simulink model "top_integrated_nanogrid"  (R2026a)
settings: Solver=ode23t  StopTime=1
values from neighbouring files (symbols this model uses):
  irradiance_day = pchip(t_coarse, irradiance_coarse, t_sim)    [flc_init.m]
  t_sim = linspace(0, 1.0, 1001)    [flc_init.m]
undefined symbols (not defined in the file or in its folder): DiscIntNeverNeededParam
libraries: fl_lib x19, nesl_utility x14, ee_lib x13, slpidlib x2, batteryecm_lib x1, fuzblock x1, eePwmGenerator x1
(part 1 of 2)
settings Model: Creator=user  LastModifiedBy=user

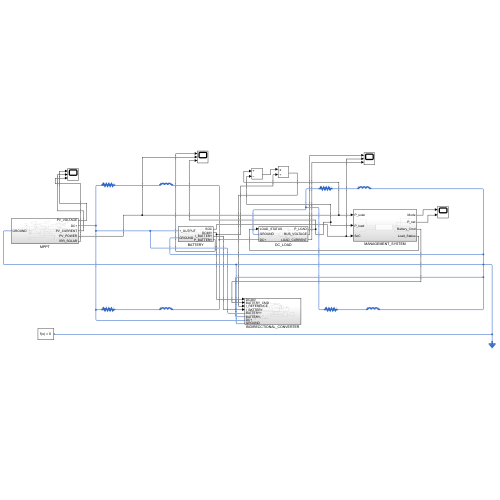
[thumbnail: Simulink's stored preview of the top-level diagram]
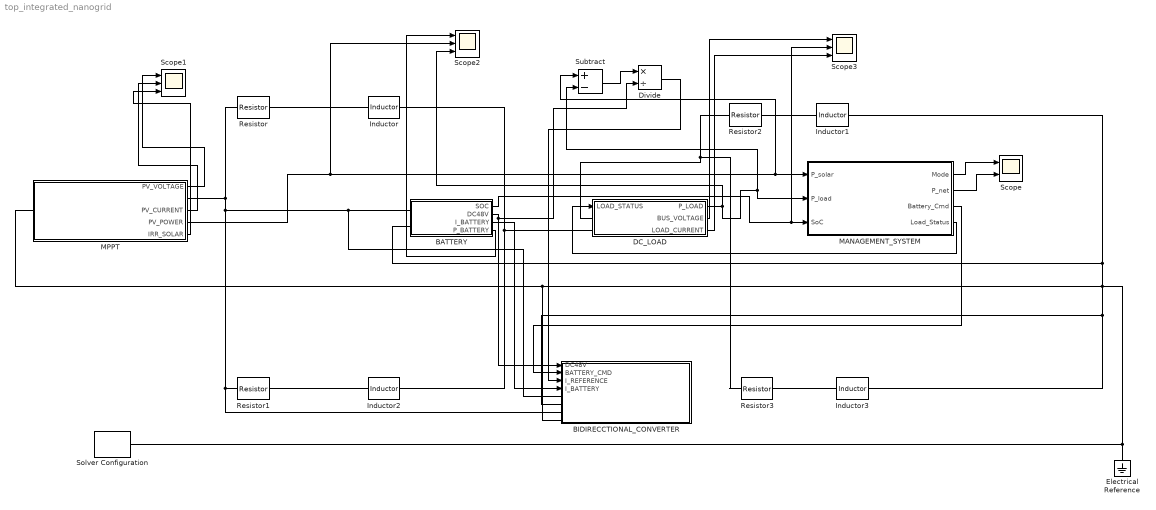
== system top_integrated_nanogrid ==
  BATTERY : Subsystem
  BIDIRECCTIONAL_CONVERTER : Subsystem
  DC_LOAD : Subsystem
  Divide : Product  Inputs=*/
  Electrical Reference : fl_lib/Electrical/Electrical Elements/Electrical Reference
  Inductor{,1..3} (4 alike) : ee_lib/Passive/Inductor  l=10e-6 H  enable_L_tol=ee.enum.toleranceApplication.none  L_tol=20  tol_distribution=ee.enum.toleranceDistribution.uniform  nSigma=4  r=0 Ohm  g=1e-9 1/Ohm  enable_operating_limits=ee.enum.enable.no  operating_limit_action=ee.enum.passive.reportOpLim.warn  max_working_current=1 A  power_rating=1 W  i_L_specify=off  i_L_priority=High  i_L=0 A  i_L_nominal_specify=off  i_L_nominal_value=1  i_L_nominal_unit=A
  MANAGEMENT_SYSTEM : Subsystem
  MPPT : Subsystem
      settings: PortSchema="{\"entries\":[{\"content\":{\"sides\":[{\"content\":{\"connectorIds\":[\"LConn1\"]},\"type\":\"ConnectorPlacement.EquallySpacedRectSide\",\"uuid\":\"0487cf4e-a869-4d13-b7ef-c52d99cbedea\"},{\"content\":{\"connectorIds\":[\"Out1\",\"RConn1\",\"Out2\",\"Out3\",\"Out4\"],\"side\":\"RIGHT\"},\"type\":\"ConnectorPlacement.EquallySpacedRectSide\",\"uuid\":\"982cd2d3-8bc2-48e7-a882-5f024f9a170e\"},{\"content\":{\"side\":\"TOP\"},\"type\":\"ConnectorPlacement.EquallySpacedRectSide\",\"uuid\":\"7eceb141-11e6-4de9-8291-895b3002810c\"}]},\"type\":\"ConnectorPlacement.EquallySpacedConnector\",\"uuid\":\"f9b56202-991f-4d6f-a8f4-53ab8bdf788c\"}],\"packageUris\":[\"http://schema.mathworks.com/mf0/Connector/R2020b\"],\"version\":\"1.0\"}"
  Resistor{,1..3} (4 alike) : fl_lib/Electrical/Electrical Elements/Resistor  R=0.23 Ohm  i_specify=off  i_priority=None  i=0 A  i_nominal_specify=off  i_nominal_value=1  i_nominal_unit=A  v_specify=off  v_priority=None  v=0 V  v_nominal_specify=off  v_nominal_value=1  v_nominal_unit=V
  Scope : Scope  NumInputPorts=2
      settings: ActiveDisplayYMinimum=-1  ActiveDisplayYMaximum=1
  Scope1 : Scope  NumInputPorts=3
      settings: ActiveDisplayYMinimum=-0.0015866090300095147  ActiveDisplayYMaximum=0.014279481270085636
  Scope2 : Scope  NumInputPorts=3
      settings: ActiveDisplayYMinimum=-1  ActiveDisplayYMaximum=1  DataLoggingVariableName=ScopeData2
  Scope3 : Scope  NumInputPorts=3
      settings: ActiveDisplayYMinimum=14.753584599444343  ActiveDisplayYMaximum=59.304634607665662  DataLoggingVariableName=ScopeData3
  Solver Configuration : nesl_utility/Solver Configuration  PhysicalDomain=network_engine_domain  SubClassName=solver  LeftPortType=input  RightPortType=generic  Tones=[]  Harmonics=[]  SimulateNoise=off  Profile=off  UseLocalSampling=off  EnableSwitchedLinearOptims=on  FrequencyDomain=off  UseCCode=off  RelTol=0.001  AbsTol=0.001  MinStep=1e-09  ToWorkspace=off  RevertToSquareIcSolve=off  NumHomotopyIterations=100  PhasorMode=off  PhasorModeNumHarmonics=1  ConsistencySolver=NEWTON_XTOL_AFTER_FTOL  CanonicalOrdering=CANONICAL  OptimizeIntermediates=OPTIMIZED  IndexReductionMethod=DerivativeReplacement  DoDC=off  ResidualTolerance=1e-09  ConsistencyTolSource=GLOBAL  ConsistencyAbsTol=0.001  ConsistencyRelTol=0.001  ConsistencyTolFactor=0.001  UseLocalSolver=off  LocalSolverChoice=NE_BACKWARD_EULER_ADVANCER  ResolveIndetEquations=on  FunctionEvalNumThread=1  LocalSolverSampleTime=0.001  DoFixedCost=off  MaxNonlinIter=3  MaxModeIter=2  ComputeImpulses=off  ImpulseIterations=2  LinearAlgebra=auto  LinearAlgebraNumThread=0  EquationFormulation=NE_TIME_EF  DelaysMemoryBudget=1024  AutomaticFiltering=on  FilteringTimeConstant=0.001  PartitionStorageMethod=AS_NEEDED  PartitionMemoryBudget=1024  PartitionMethod=ROBUST  MultibodyUseLocalSolver=off  MultibodyLocalSolverChoice=ODE1  MultibodyLocalSolverSampleTime=0.001
  Subtract : Sum  Inputs=+-
  wires:
  BATTERY/1(SOC) -> Scope3/2, MANAGEMENT_SYSTEM/3(SoC)
  MANAGEMENT_SYSTEM/4(Load_Status) -> DC_LOAD/1(LOAD_STATUS)
  MANAGEMENT_SYSTEM/1(Mode) -> Scope/1
  MANAGEMENT_SYSTEM/2(P_net) -> Scope/2
  MANAGEMENT_SYSTEM/3(Battery_Cmd) -> BIDIRECCTIONAL_CONVERTER/2(BATTERY_CMD)
  MPPT/3(PV_POWER) -> Scope2/2, Subtract/1, MANAGEMENT_SYSTEM/1(P_solar)
  DC_LOAD/1(P_LOAD) -> Subtract/2, MANAGEMENT_SYSTEM/2(P_load), Scope2/3
  Subtract/1 -> Divide/1
  BATTERY/2(DC48V) -> Divide/2, BIDIRECCTIONAL_CONVERTER/1(DC48V)
  Divide/1 -> BIDIRECCTIONAL_CONVERTER/3(I_REFERENCE)
  BATTERY/3(I_BATTERY) -> BIDIRECCTIONAL_CONVERTER/4(I_BATTERY)
  MPPT/1(PV_VOLTAGE) -> Scope1/1
  MPPT/2(PV_CURRENT) -> Scope1/2
  MPPT/4(IRR_SOLAR) -> Scope1/3
  BATTERY/4(P_BATTERY) -> Scope2/1
  DC_LOAD/2(BUS_VOLTAGE) -> Scope3/1
  DC_LOAD/3(LOAD_CURRENT) -> Scope3/3
  connections:
  Resistor/RConn1 -- Inductor/LConn1
  Resistor2/RConn1 -- Inductor1/LConn1
  Resistor1/RConn1 -- Inductor2/LConn1
  Resistor3/RConn1 -- Inductor3/LConn1
  BATTERY/LConn1 -- BIDIRECCTIONAL_CONVERTER/LConn1 -- MPPT/RConn1 -- Resistor/LConn1 -- BIDIRECCTIONAL_CONVERTER/LConn3 -- Resistor1/LConn1
  Inductor1/RConn1 -- BIDIRECCTIONAL_CONVERTER/LConn2 -- Inductor3/RConn1 -- BIDIRECCTIONAL_CONVERTER/LConn4 -- MPPT/LConn1 -- Solver Configuration/RConn1 -- Electrical Reference/LConn1 -- BATTERY/LConn2
  Inductor/RConn1 -- Inductor2/RConn1 -- DC_LOAD/LConn2
  Resistor2/LConn1 -- Resistor3/LConn1 -- DC_LOAD/LConn1

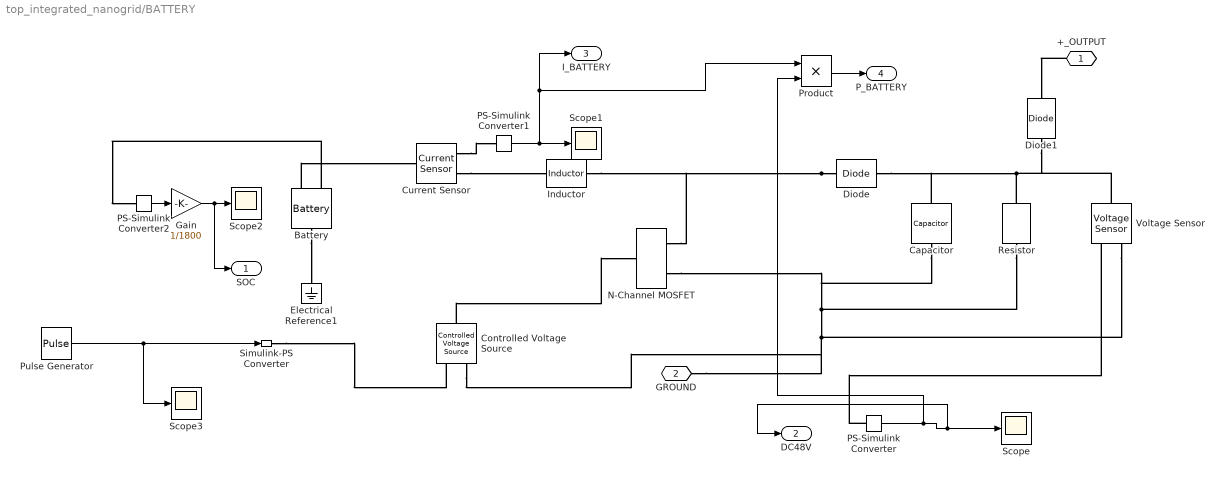
== system top_integrated_nanogrid/BATTERY ==
  Battery : batteryecm_lib/Battery  Vnom=24 V  prm_dir=simscape.enum.battery.prm_dir.enabled  R1_dis=0.001 Ohm  R1_ch=0.001 Ohm  R1=0.001 Ohm  prm_AH=simscape.enum.battery.prm_AH.finite  AH=50 A*hr  V1=11.5 V  AH1=25 A*hr  prm_R2=simscape.enum.battery.prm_R2.disabled  R2=2000 Ohm  Tmeas=298.15 K  charge_measurement_port=simscape.enum.battery.enable.yes  prm_dyn=simscape.enum.battery.prm_dyn.off  Rp1=0.005 Ohm  tau1=30 s  Rp2=0.005 Ohm  tau2=30 s  Rp3=0.005 Ohm  tau3=30 s  Rp4=0.005 Ohm  tau4=30 s  Rp5=0.005 Ohm  tau5=30 s  prm_fade=simscape.enum.battery.prm_fade.disabled  N_fade=100  AH_fade=45 A*hr  R1_fade=2.02 Ohm  R1_ch_fade=2.02 Ohm  V1_fade=10.35 V  prm_age=simscape.enum.battery.prm_age.disabled  prm_age_OCV=simscape.enum.battery.prm_age_OCV.OCV  OCV_age=0.9  SOC_age=60  Tmeas_age=298.15 K  delta_time_age_vec=[0] d  temperature_age_vec=[273] K  OCV_scaling_age=2.2134e6  OCV_offset_age=1.632e6  temp_exp_age=0.515833569 V  t_exp_age=0.75  Vnom_T2=12 V  R1_T2=2.2 Ohm  R1_T2_dis=2.2 Ohm  R1_T2_ch=2.2 Ohm  V1_T2=11.4 V  R2_T2=2200 Ohm  Rp1_T2=0.005 Ohm  tau1_T2=30 s  Rp2_T2=0.005 Ohm  tau2_T2=30 s  Rp3_T2=0.005 Ohm  tau3_T2=30 s  Rp4_T2=0.005 Ohm  tau4_T2=30 s  Rp5_T2=0.005 Ohm  tau5_T2=30 s  Tmeas2=273.15 K  thermal_port=simscape.enum.thermaleffects.omit  thermal_mass=30000 J/K  i_specify=off  i_priority=None  i=0 A  i_nominal_specify=off  i_nominal_value=1  i_nominal_unit=A  v_specify=off  v_priority=None  v=0 V  v_nominal_specify=off  v_nominal_value=1  v_nominal_unit=V  charge_specify=off  charge_priority=High  charge=50 A*hr  charge_nominal_specify=off  charge_nominal_value=1  charge_nominal_unit=A*hr  num_cycles_specify=off  num_cycles_priority=High  num_cycles=0  num_cycles_nominal_specify=off  num_cycles_nominal_value=1  num_cycles_nominal_unit=1  temperature_specify=off  temperature_priority=High  temperature=298.15 K  temperature_nominal_specify=off  temperature_nominal_value=1  temperature_nominal_unit=K
  Capacitor : fl_lib/Electrical/Electrical Elements/Capacitor  c=220 uF  r=1e-6 Ohm  g=0 1/Ohm  i_specify=off  i_priority=None  i=0 A  i_nominal_specify=off  i_nominal_value=1  i_nominal_unit=A  v_specify=off  v_priority=None  v=0 V  v_nominal_specify=off  v_nominal_value=1  v_nominal_unit=V  vc_specify=off  vc_priority=High  vc=0 V  vc_nominal_specify=off  vc_nominal_value=1  vc_nominal_unit=V
  Controlled Voltage Source : fl_lib/Electrical/Electrical Sources/Controlled Voltage Source
  Current Sensor : fl_lib/Electrical/Electrical Sensors/Current Sensor
  Diode : fl_lib/Electrical/Electrical Elements/Diode  Vf=0.7 V  Ron=0.001 Ohm  Goff=1e-8 1/Ohm  i_specify=off  i_priority=None  i=0 A  i_nominal_specify=off  i_nominal_value=1  i_nominal_unit=A  v_specify=off  v_priority=None  v=0 V  v_nominal_specify=off  v_nominal_value=1  v_nominal_unit=V
  Diode1 : ee_lib/Semiconductors & Converters/Diode  ModelType=ee.enum.diode.modelType.pwl  TableType=ee.enum.diode.tableType.IfMat  IfMat=[.07, .12, .19, 1.75, 4.24, 7.32, 11.2; .16, .3, .72, 2.14, 5.02, 8.35, 13.12] A  VfMat=[.9, 1.15, 1.25, 1.5, 1.75, 2.17, 2.6, 2.85; .58, .68, .75, 1.1, 1.38, 1.77, 2.27, 2.7] V  TjVec=[25, 125] degC  VfVec=[.5, .7, .9, 1.3, 1.7, 2.1, 2.5] V  IfVec=[.1, .2, .5, 1, 2, 4, 7, 10] A  IrMat=[1e-06, 2e-06, 5e-06, 1e-05, 2.5e-05, 5e-05, .0001; 2e-06, 5e-06, 1e-05, 4e-05, 8e-05, .0002, .0005] A  VrMat=[10, 100, 200, 250, 300, 325, 350; 10, 70, 160, 220, 270, 300, 320] V  VrVec=[10, 20, 40, 50, 70, 80, 100] V  IrVec=[1e-06, 2e-06, 5e-06, 1e-05, 2e-05, 5e-05, .0001] A  Vf=0.6 V  Ron=0.3 Ohm  Goff=1e-8 S  prmExp=ee.enum.diode.expParam.useTwo  I12=[.0137, .545] A  V12=[.6, .7] V  RS=0 Ohm  Tmeas=298.15 K  IS=1e-12 A  ec=1  I1=0.0137 A  V1=0.6 V  N_series=1  N_parallel=1  ZenerEnable=false  Rz=0.3 Ohm  BV=30 V  C_param=ee.enum.diode.capParam.fixed  CJ=0 pF  CJ0=5 pF  Vvec=[.1, 10, 100] V  Cvec=[3.5, 1, .4] pF  VJ=1 V  Mgrad=0.5  FC=0.5  Q_param=ee.enum.diode.recoveryParam.off  iRM=-7.15 A  iF=4 A  didt=-750 A/us  trr_factor=3  trr=115 ns  Qrr=150 nA*s  Vr=-600 V  Ls=150 nH  Erec=0.03 J  TT=50 ns  tau=100 ns  T_param=ee.enum.diode.temperatureParam.off  Tdevice=298.15 K  I1_T2=0.245 A  V1_T2=0.5 V  IS_T2=1.25e-7 A  Tmeas2=125 degC  XTI_param=ee.enum.diode.xtiParam.pn  XTI=3  EG_param=ee.enum.diode.egapParam.material_si  EG=1.11 eV  dBVdT=0 V/K  enable_fault_input=simscape.enum.onoff.off  i_specify=off  i_priority=None  i=0 A  i_nominal_specify=off  i_nominal_value=1  i_nominal_unit=A  v_specify=off  v_priority=None  v=0 V  v_nominal_specify=off  v_nominal_value=1  v_nominal_unit=V  v_capacitor_specify=off  v_capacitor_priority=None  v_capacitor=0 V  v_capacitor_nominal_specify=off  v_capacitor_nominal_value=1  v_capacitor_nominal_unit=V  Qj_specify=off  Qj_priority=High  Qj=0 C  Qj_nominal_specify=off  Qj_nominal_value=1  Qj_nominal_unit=C  i_diode_specify=off  i_diode_priority=None  i_diode=0 A  i_diode_nominal_specify=off  i_diode_nominal_value=1  i_diode_nominal_unit=A  v_diode_specify=off  v_diode_priority=None  v_diode=0 V  v_diode_nominal_specify=off  v_diode_nominal_value=1  v_diode_nominal_unit=V  i_capacitor_specify=off  i_capacitor_priority=None  i_capacitor=0 A  i_capacitor_nominal_specify=off  i_capacitor_nominal_value=1  i_capacitor_nominal_unit=A  fidelity_level=ee.enum.diode.fidelity.includeChargeDyn  rec_loss_model=ee.enum.diode.reverseRecoveryModelTabulateUpTo3D.fixed  ErecVal=0 J  scaleWithIandV=true  ErecMat=zeros(2, 3) J  ErecMat3D=zeros(2, 3, 2) J  TjrecVec=[298.15, 398.15] K  IfrecVec=[.1, 1, 10] A  IrecVal=10 A  VrecVal=10 V  VrecVec=[0, 100] V  tFilter=1 / 1000 / 100 s  thermal_network_parameterization=ee.enum.thermalNetworkTopology.junctionCase  Rth=[0, 10] K/W  Rth_Cauer=[1, 3, 10] K/W  Rth_Foster=[.08, .14, .22, .16] K/W  thermal_mass_parameterization=ee.enum.thermalNetwork.timeconstant  thermal_mass=[0, 1] J/K  thermal_mass_Cauer=[.1, .3, 1] J/K  thermal_mass_Foster=[.001, .005, .05, .5] J/K  thermal_time_constant=[0, 10] s  thermal_time_constant_Cauer=[1, 3, 10] s  thermal_time_constant_Foster=[7e-05, .0007, .01, .08] s  thermal_mass_initial_temperatures=[25, 25] degC  thermal_mass_initial_temperatures_Cauer=[25, 25, 25] degC  junction_thermal_mass=0.01 J/K  Tvec_initial_Foster=[25, 25, 25, 25] degC  no_thermal_network=0  junction_temperature_specify=off  junction_temperature_priority=None  junction_temperature=25 degC  junction_temperature_nominal_specify=off  junction_temperature_nominal_value=1  junction_temperature_nominal_unit=degC
  Electrical Reference1 : fl_lib/Electrical/Electrical Elements/Electrical Reference
  Gain : Gain  Gain=1/1800
  Inductor : ee_lib/Passive/Inductor  l=100 uH  enable_L_tol=ee.enum.toleranceApplication.none  L_tol=20  tol_distribution=ee.enum.toleranceDistribution.uniform  nSigma=4  r=0 Ohm  g=1e-9 1/Ohm  enable_operating_limits=ee.enum.enable.no  operating_limit_action=ee.enum.passive.reportOpLim.warn  max_working_current=1 A  power_rating=1 W  i_L_specify=off  i_L_priority=High  i_L=0 A  i_L_nominal_specify=off  i_L_nominal_value=1  i_L_nominal_unit=A
  N-Channel MOSFET : ee_lib/Semiconductors & Converters/N-Channel MOSFET  paramTerminal=ee.enum.mosfet.numberOfTerminals.three  parameterization=ee.enum.mosfet.parameterization.datasheet  Beta=5.0 A/V^2  Rds=0.01 mOhm  Id=6.0 A  Vgs=10 V  Vth=1.7 V  Vth0=1.7 V  lam=0 1/V  gamma_vth=0.5 V^(1/2)  phib=0.5 V  Vth1=1.9071 V  Vbs1=-1 V  Vth2=2.066 V  Vbs2=-2 V  Tmeas=25 degC  Vgs_vec=[-1, -.5, 2, 3, 4, 5] V  Vds_vec=[0, 2, 4, 8, 12, 16, 20] V  Vbs_vec=[0, -4, -6, -12] V  T_vec=[25, 125] degC  Vth_vec=[.4, 1.2, 1.4, 1.45] V  Vth_mat=[.4, .35; 1.2, 1.15; 1.4, 1.35; 1.45, 1.4] V  Ids_mat=[0, 0, 0, 0, 0, 0, 0; 0, 0, 0, 0, 0, 0, 0; 0, .003, .0038, .0043, .0046, .0048, .0049; 0, .0055, .008, .009, .0095, .01, .0101; 0, .0115, .016, .018, .019, .0195, .02; 0, .0152, .0225, .0265, .028, .0295, .03] A  Ids_mat0=[0, 0, 0, 0, 0, 0, 0; 0, 0, 0, 0, 0, 0, 0; 0, .003, .0038, .0043, .0046, .0048, .0049; 0, .0055, .008, .009, .0095, .01, .0101; 0, .0115, .016, .018, .019, .0195, .02; 0, .0152, .0225, .0265, .028, .0295, .03] A  Ids_mat_3D=zeros(6, 7, 2) A  Ids_mat_3D0=zeros(6, 7, 2) A  IV_table_symmetry=ee.enum.mosfet.symmetricNIV.no  RS=0.001 mOhm  RD=0.001 mOhm  RB=0.001 Ohm  LeadRs=0 Ohm  LeadRd=0 Ohm  LeadRg=0 Ohm  LeadRb=0 Ohm  LS=0 nH  LD=0 nH  LG=0 nH  LB=0 nH  C_param=ee.enum.mosfet.capacitanceParam.fixedciss  C_GS=270 pF  C_GD=80 pF  C_GB=0 pF  C_DS=0 pF  C_iss=350 pF  C_rss=80 pF  C_oss=0 pF  C_iss_vec=[720, 700, 590, 470, 390, 310] pF  C_rss_vec=[450, 400, 300, 190, 95, 55] pF  C_oss_vec=[900, 810, 690, 420, 270, 170] pF  C_GS_vec=[270, 300, 290, 280, 295, 255] pF  C_GD_vec=[450, 400, 300, 190, 95, 55] pF  C_GB_vec=[270, 300, 290, 280, 295, 255] pF  C_Vgs_vec=0 V  C_DS_vec=[450, 410, 390, 230, 175, 115] pF  C_Vds_vec=[.1, .3, 1, 3, 10, 30] V  V_GS_for_cap_data=0 V  charge_linearity_param=ee.enum.mosfet.cgdLinearity.constant  C_OX=200 pF  V_C_OX=-0.5 V  charge_linearity_param_vgb=ee.enum.mosfet.cgbLinearity.instantly  charge_linearity_param_with_vgb=ee.enum.mosfet.cgbLinearityWithSeparateCgb.instantly  Di_param=ee.enum.mosfet.diodeParam.no  IsDiode=1e-12 A  Vbi=0.6 V  n=1  Cj0Diode=0 pF  TT=50e-9 s  Tmeas_dio=25 degC  TableTypeNoT=ee.enum.mosfet.tableType.IfMat  TableType=ee.enum.diode.tableType.IfMat  IfVec=[.07, .12, .19, 1.75, 4.24, 7.32, 11.2] A  IfMat=[.07, .12, .19, 1.75, 4.24, 7.32, 11.2; .16, .3, .72, 2.14, 4.02, 6.35, 9.12] A  VfVecV=[.9, 1.15, 1.25, 1.5, 1.75, 2.17, 2.6, 2.85] V  VfMatV=[.9, 1.15, 1.25, 1.5, 1.75, 2.17, 2.6, 2.85; .58, .68, .75, 1.1, 1.38, 1.77, 2.27, 2.7] V  TjVec=[25, 125] degC  VfVec=[.5, .7, .9, 1.3, 1.7, 2.1, 2.5] V  IfVecV=[.1, .2, .5, 1, 2, 4, 7, 10] A  diode_Goff=1e-12 1/Ohm  prmDatasheet=ee.enum.temperatureParameterization.none  prmEquCoeff=ee.enum.temperatureParameterization.none  dVth_dT=-6 mV/K  dVth0_dT=-6 mV/K  Rds_T2=0.037 Ohm  BEXDatasheet=-1.5  BEXEquCoeff=-1.5  etaisDatasheet=3  etaisEquCoeff=3  Tmeas2=125 degC  etaisTabulated=3  TdeviceDatasheet=25 degC  TdeviceEquCoeff=25 degC  TdeviceTabulated=25 degC  i_g_specify=off  i_g_priority=None  i_g=0 A  i_g_nominal_specify=off  i_g_nominal_value=1  i_g_nominal_unit=A  i_d_specify=off  i_d_priority=None  i_d=0 A  i_d_nominal_specify=off  i_d_nominal_value=1  i_d_nominal_unit=A  i_b_specify=off  i_b_priority=None  i_b=0 A  i_b_nominal_specify=off  i_b_nominal_value=1  i_b_nominal_unit=A  voltage_gs_specify=off  voltage_gs_priority=None  voltage_gs=0 V  voltage_gs_nominal_specify=off  voltage_gs_nominal_value=1  voltage_gs_nominal_unit=V  voltage_ds_specify=off  voltage_ds_priority=None  voltage_ds=0 V  voltage_ds_nominal_specify=off  voltage_ds_nominal_value=1  voltage_ds_nominal_unit=V  voltage_bs_specify=off  voltage_bs_priority=None  voltage_bs=0 V  voltage_bs_nominal_specify=off  voltage_bs_nominal_value=1  voltage_bs_nominal_unit=V  v_Cgs_specify=off  v_Cgs_priority=High  v_Cgs=0 V  v_Cgs_nominal_specify=off  v_Cgs_nominal_value=1  v_Cgs_nominal_unit=V  v_Cds_specify=off  v_Cds_priority=High  v_Cds=0 V  v_Cds_nominal_specify=off  v_Cds_nominal_value=1  v_Cds_nominal_unit=V  v_Cbs_specify=off  v_Cbs_priority=High  v_Cbs=0 V  v_Cbs_nominal_specify=off  v_Cbs_nominal_value=1  v_Cbs_nominal_unit=V  thermal_network_parameterization=ee.enum.thermalNetworkTopology.junctionCase  Rth=[0, 10] K/W  Rth_Cauer=[1, 3, 10] K/W  Rth_Foster=[.08, .14, .22, .16] K/W  thermal_mass_parameterization=ee.enum.thermalNetwork.timeconstant  thermal_mass=[0, 1] J/K  thermal_mass_Cauer=[.1, .3, 1] J/K  thermal_mass_Foster=[.001, .005, .05, .5] J/K  thermal_time_constant=[0, 10] s  thermal_time_constant_Cauer=[1, 3, 10] s  thermal_time_constant_Foster=[7e-05, .0007, .01, .08] s  thermal_mass_initial_temperatures=[25, 25] degC  thermal_mass_initial_temperatures_Cauer=[25, 25, 25] degC  Tvec_initial_Foster=[25, 25, 25, 25] degC  betaref=18 A/V^2  Vfbref=-1.1 V  gamma=3.5 V^(1/2)  phib2ref=1 V  thesatref=0.4 1/V  alpha=0  Vp=5e-2 V  thesrref=0 1/V  m=8  Tref=25 degC  Rsref=2e-3 Ohm  Rdref=0.17 Ohm  Rgref=8.4 Ohm  Rbref=2e-3 Ohm  Cox=1500 pF  Cgso=100 pF  Cgdo=14 pF  Isref=5.2e-13 A  Cj0=480 pF  Tprm=ee.enum.temperatureParameterization.none  etabet=1.3  Stvfb=5e-4 V/K  Stphib=-8.5e-4 V/K  etasat=1.04  etasr=0.65  etar=0.95  etais=3  Tsim=25 degC  Ig_specify=off  Ig_priority=None  Ig=0 A  Ig_nominal_specify=off  Ig_nominal_value=1  Ig_nominal_unit=nA  Ids_specify=off  Ids_priority=None  Ids=0 A  Ids_nominal_specify=off  Ids_nominal_value=1  Ids_nominal_unit=A  Ib_specify=off  Ib_priority=None  Ib=0 A  Ib_nominal_specify=off  Ib_nominal_value=1  Ib_nominal_unit=uA  V_gs_specify=off  V_gs_priority=None  V_gs=0 V  V_gs_nominal_specify=off  V_gs_nominal_value=1  V_gs_nominal_unit=V  V_ds_specify=off  V_ds_priority=None  V_ds=0 V  V_ds_nominal_specify=off  V_ds_nominal_value=1  V_ds_nominal_unit=V  V_bs_specify=off  V_bs_priority=None  V_bs=0 V  V_bs_nominal_specify=off  V_bs_nominal_value=1  V_bs_nominal_unit=V  QGoverCox_specify=off  QGoverCox_priority=None  QGoverCox=0 V  QGoverCox_nominal_specify=off  QGoverCox_nominal_value=1  QGoverCox_nominal_unit=V  QDoverCox_specify=off  QDoverCox_priority=None  QDoverCox=0 V  QDoverCox_nominal_specify=off  QDoverCox_nominal_value=1  QDoverCox_nominal_unit=V  QBoverCox_specify=off  QBoverCox_priority=None  QBoverCox=0 V  QBoverCox_nominal_specify=off  QBoverCox_nominal_value=1  QBoverCox_nominal_unit=V  T0=[25, 25] degC  T0_Cauer=[25, 25, 25] degC
  PS-Simulink Converter : nesl_utility/PS-Simulink Converter  PhysicalDomain=network_engine_domain  SubClassName=ps_output  LeftPortType=input  RightPortType=output  PseudoPeriodic=off  Frequencies=[]  VectorFormat=inherit  Unit=inherit  AffineConversion=off
  PS-Simulink Converter1 : nesl_utility/PS-Simulink Converter  PhysicalDomain=network_engine_domain  SubClassName=ps_output  LeftPortType=input  RightPortType=output  PseudoPeriodic=off  Frequencies=[]  VectorFormat=inherit  Unit=inherit  AffineConversion=off
  PS-Simulink Converter2 : nesl_utility/PS-Simulink Converter  PhysicalDomain=network_engine_domain  SubClassName=ps_output  LeftPortType=input  RightPortType=output  PseudoPeriodic=off  Frequencies=[]  VectorFormat=inherit  Unit=inherit  AffineConversion=off
  Product : Product
  Pulse Generator : DiscretePulseGenerator  PulseType=Time based  Amplitude=10  Period=1e-4  PulseWidth=52  PhaseDelay=1e-5
  Resistor : fl_lib/Electrical/Electrical Elements/Resistor  R=10 Ohm  i_specify=off  i_priority=None  i=0 A  i_nominal_specify=off  i_nominal_value=1  i_nominal_unit=A  v_specify=off  v_priority=None  v=0 V  v_nominal_specify=off  v_nominal_value=1  v_nominal_unit=V
  Scope{,1..3} (4 alike) : Scope
      Scope settings: ActiveDisplayYMinimum=-7.926026759259857  ActiveDisplayYMaximum=71.334240833338725  DataLoggingVariableName=ScopeData17
      Scope1 settings: ActiveDisplayYMinimum=-10.159654600356284  ActiveDisplayYMaximum=91.182954758097466  DataLoggingVariableName=ScopeData18
      Scope2 settings: ActiveDisplayYMinimum=99.999790390076058  ActiveDisplayYMaximum=100.00002328999156  DataLoggingVariableName=ScopeData19
      Scope3 settings: ActiveDisplayYMinimum=-1.2499999999999998  ActiveDisplayYMaximum=11.25  DataLoggingVariableName=ScopeData20
  Simulink-PS Converter : nesl_utility/Simulink-PS Converter  PhysicalDomain=network_engine_domain  SubClassName=ps_input  LeftPortType=input  RightPortType=output  PseudoPeriodic=off  Frequencies=[]  NoiseDistribution=none  NoiseParameters=[]  Unit=1  AffineConversion=off  FilteringAndDerivatives=provide  SimscapeFilterOrder=1  InputFilterTimeConstant=0.001  UdotUserProvided=0
  Voltage Sensor : fl_lib/Electrical/Electrical Sensors/Voltage Sensor
  +_OUTPUT : PMIOPort  Side=Left
  GROUND : PMIOPort  Port=2  Side=Left
  SOC : Outport
  DC48V : Outport  Port=2
  I_BATTERY : Outport  Port=3
  P_BATTERY : Outport  Port=4
  wires:
  PS-Simulink Converter/1 -> Product/2, DC48V/1, Scope/1
  PS-Simulink Converter2/1 -> Gain/1
  PS-Simulink Converter1/1 -> Product/1, I_BATTERY/1, Scope1/1
  Gain/1 -> SOC/1, Scope2/1
  Pulse Generator/1 -> Scope3/1, Simulink-PS Converter/1
  Product/1 -> P_BATTERY/1
  connections:
  Voltage Sensor/RConn2 -- Controlled Voltage Source/RConn2 -- GROUND/RConn1 -- N-Channel MOSFET/RConn2 -- Capacitor/RConn1 -- Resistor/RConn1
  Resistor/LConn1 -- Voltage Sensor/LConn1 -- Diode1/LConn1 -- Diode/RConn1 -- Capacitor/LConn1
  Diode/LConn1 -- Inductor/RConn1 -- N-Channel MOSFET/RConn1
  Battery/LConn2 -- PS-Simulink Converter2/LConn1
  PS-Simulink Converter/LConn1 -- Voltage Sensor/RConn1
  Current Sensor/RConn2 -- Inductor/LConn1
  Battery/RConn1 -- Electrical Reference1/LConn1
  Current Sensor/RConn1 -- PS-Simulink Converter1/LConn1
  Battery/LConn1 -- Current Sensor/LConn1
  Simulink-PS Converter/RConn1 -- Controlled Voltage Source/RConn1
  Controlled Voltage Source/LConn1 -- N-Channel MOSFET/LConn1
  +_OUTPUT/RConn1 -- Diode1/RConn1

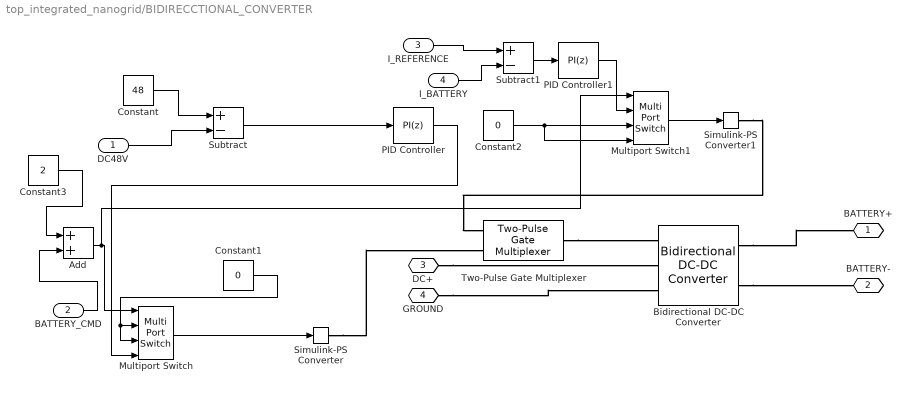
== system top_integrated_nanogrid/BIDIRECCTIONAL_CONVERTER ==
  DC48V : Inport
  BATTERY_CMD : Inport  Port=2
  I_REFERENCE : Inport  Port=3
  I_BATTERY : Inport  Port=4
  Add : Sum
  Bidirectional DC-DC Converter : ee_lib/Semiconductors & Converters/Converters/Bidirectional DC-DC Converter  fidelity_option=ee.enum.converters.fidelity.equivalent_pwm  device_type=ee.enum.converters.switchingdevice.ideal  Vf=0.8 V  Ron=0.001 Ohm  Rds=0.001 Ohm  Goff=1e-5 1/Ohm  Vth=6 V  Vgt=1 V  Vgt_off=-1 V  Ih=1 A  K=0  diode_param=ee.enum.converters.diode.nodynamics  diode_Vf=0.8 V  diode_Ron=0.001 Ohm  diode_Goff=1e-5 1/Ohm  diode_C=50 nF  diode_iRM=-235 A  diode_iF=300 A  diode_idot=-50 A/us  diode_trr_param=ee.enum.converters.diodetrr.trr_factor  diode_trr_factor=3  diode_trr=15 us  diode_Qrr=1500 s*uA  L=1e-3 H  Rl=0.01 Ohm  C1=470 uF  C2=1000 uF  R1=1e-3 Ohm  R2=1e-3 Ohm  snubber_type=ee.enum.converters.snubber.exclude  Cs=1e-7 F  Rs=0.1 Ohm  iL_specify=off  iL_priority=High  iL=0 A  iL_nominal_specify=off  iL_nominal_value=1  iL_nominal_unit=A  vc1_specify=off  vc1_priority=High  vc1=0 V  vc1_nominal_specify=off  vc1_nominal_value=1  vc1_nominal_unit=V  vc2_specify=off  vc2_priority=High  vc2=0 V  vc2_nominal_specify=off  vc2_nominal_value=1  vc2_nominal_unit=V  device_type_hv=ee.enum.converters.switchingdevice.ideal  Vf_hv=0.8 V  Ron_hv=0.001 Ohm  Rds_hv=0.001 Ohm  Goff_hv=1e-5 1/Ohm  Vth_hv=6 V  Vgt_hv=1 V  Vgt_off_hv=-1 V  Ih_hv=1 A  device_type_lv=ee.enum.converters.switchingdevice.ideal  Vf_lv=0.8 V  Ron_lv=0.001 Ohm  Rds_lv=0.001 Ohm  Goff_lv=1e-5 1/Ohm  Vth_lv=6 V  Vgt_lv=1 V  Vgt_off_lv=-1 V  Ih_lv=1 A  T_L1=0.03 H  T_L2=0.03 H  T_k=0.9  snubber_type_hv=ee.enum.converters.snubber.exclude  Cs_hv=1e-7 F  Rs_hv=0.1 Ohm  snubber_type_lv=ee.enum.converters.snubber.exclude  Cs_lv=1e-7 F  Rs_lv=0.1 Ohm  iL1_specify=off  iL1_priority=High  iL1=0 A  iL1_nominal_specify=off  iL1_nominal_value=1  iL1_nominal_unit=A  iL2_specify=off  iL2_priority=High  iL2=0 A  iL2_nominal_specify=off  iL2_nominal_value=1  iL2_nominal_unit=A  hysteresisCurrent=0.0005 A
  Constant : Constant  Value=48
  Constant1 : Constant  Value=0
  Constant2 : Constant  Value=0
  Constant3 : Constant  Value=2
  Multiport Switch : MultiPortSwitch  SaturateOnIntegerOverflow=off  InputSameDT=off
  Multiport Switch1 : MultiPortSwitch  SaturateOnIntegerOverflow=off  InputSameDT=off
  PID Controller : slpidlib/PID Controller  Controller=PI  Form=Parallel  TimeDomain=Discrete-time  UseExternalTs=off  SampleTime=-1  IntegratorMethod=Forward Euler  FilterMethod=Forward Euler  ControllerParametersSource=internal  P=0.1  I=10  UseKiTs=off  D=0  UseExternalDerivativeSource=off  N=100  UseFilter=on  TunerSelectOption=Transfer Function Based (PID Tuner App)  InitialConditionSource=internal  InitialConditionForIntegrator=0  InitialConditionForFilter=0  DifferentiatorICPrevScaledInput=0  ExternalReset=none  TrackingMode=off  Kt=1  LimitOutput=on  SatLimitsSource=internal  UpperSaturationLimit=0.9  LowerSaturationLimit=0  LinearizeAsGain=on  AntiWindupMode=none  Kb=1  LimitIntegrator=off  UpperIntegratorSaturationLimit=inf  LowerIntegratorSaturationLimit=-inf  POutMin=[]  POutMax=[]  IOutMin=[]  IOutMax=[]  DOutMin=[]  DOutMax=[]  NOutMin=[]  NOutMax=[]  SumOutMin=[]  SumOutMax=[]  SaturationOutMin=[]  SaturationOutMax=[]  PParamMin=[]  PParamMax=[]  IParamMin=[]  IParamMax=[]  DParamMin=[]  DParamMax=[]  NParamMin=[]  NParamMax=[]  KbParamMin=[]  KbParamMax=[]  KtParamMin=[]  KtParamMax=[]  KbOutMin=[]  KbOutMax=[]  KtOutMin=[]  KtOutMax=[]  IntegratorOutMin=[]  IntegratorOutMax=[]  FilterOutMin=[]  FilterOutMax=[]  SumI1OutMin=[]  SumI1OutMax=[]  SumI2OutMin=[]  SumI2OutMax=[]  SumI3OutMin=[]  SumI3OutMax=[]  SumI4OutMin=[]  SumI4OutMax=[]  SumDOutMin=[]  SumDOutMax=[]  DifferentiatorOutMin=[]  DifferentiatorOutMax=[]  FilterDiffOutCoefMin=[]  FilterDiffOutCoefMax=[]  ReciprocalOutMin=[]  ReciprocalOutMax=[]  SumDenOutMin=[]  SumDenOutMax=[]  SumNumOutMin=[]  SumNumOutMax=[]  DivideOutMin=[]  DivideOutMax=[]  UdiffTsProdOutMin=[]  UdiffTsProdOutMax=[]  NTsProdOutMin=[]  NTsProdOutMax=[]  UintegralTsProdOutMin=[]  UintegralTsProdOutMax=[]  UngainTsProdOutMin=[]  UngainTsProdOutMax=[]  ClampingZeroOutDataTypeStr=Inherit: Inherit via back propagation  ClampingZeroOutMin=[]  ClampingZeroOutMax=[]  FilterDenConstantOutDataTypeStr=Inherit: Inherit via back propagation  FilterDenConstantOutMin=[]  FilterDenConstantOutMax=[]  PCopyOutDataTypeStr=Inherit: Inherit via back propagation  PCopyOutMin=[]  PCopyOutMax=[]  NCopyOutDataTypeStr=Inherit: Inherit via back propagation  NCopyOutMin=[]  NCopyOutMax=[]  IntegratorContinuousStateAttributes=''  IntegratorStateMustResolveToSignalObject=off  IntegratorRTWStateStorageClass=Auto  FilterContinuousStateAttributes=''  FilterStateMustResolveToSignalObject=off  FilterRTWStateStorageClass=Auto  ParallelPVariant=InternalParameters  IdealPVariant=Disabled  IVariant=InternalParameters  DVariant=Disabled  IntegratorVariant=Discrete  SatVariant=Enabled  AWVariant=Passthrough  PCopyVariant=Disabled  TRVariant=Disabled  FdbkBlocksVariant=Forward  IdealPFdbkVariant=Disabled  SatFdbkVariant=Disabled  DerivativeFilterVariant=Disabled  NVariant=Disabled  NCopyVariant=Disabled_SignalSpec  FilterICVariant=Disabled  IntegratorICVariant=InternalICs  ExternalResetVariant=Disabled  TRSumVariant=Passthrough  SumFdbkVariant=Disabled  SumVariant=Sum_PI  TsampFilterVariant=InternalTs  TsampNgainVariant=Passthrough  TsampIntegralVariant=Disabled_SignalSpec  ExternalSaturationOutDataTypeStr=Inherit: Same as second input  DerivativeSourceVariant=Disabled  PreIntVariant=InternalPreInt
  PID Controller1 : slpidlib/PID Controller  Controller=PI  Form=Parallel  TimeDomain=Discrete-time  UseExternalTs=off  SampleTime=-1  IntegratorMethod=Forward Euler  FilterMethod=Forward Euler  ControllerParametersSource=internal  P=0.1  I=10  UseKiTs=off  D=0  UseExternalDerivativeSource=off  N=100  UseFilter=on  TunerSelectOption=Transfer Function Based (PID Tuner App)  InitialConditionSource=internal  InitialConditionForIntegrator=0  InitialConditionForFilter=0  DifferentiatorICPrevScaledInput=0  ExternalReset=none  TrackingMode=off  Kt=1  LimitOutput=on  SatLimitsSource=internal  UpperSaturationLimit=0.9  LowerSaturationLimit=0  LinearizeAsGain=on  AntiWindupMode=none  Kb=1  LimitIntegrator=off  UpperIntegratorSaturationLimit=inf  LowerIntegratorSaturationLimit=-inf  POutMin=[]  POutMax=[]  IOutMin=[]  IOutMax=[]  DOutMin=[]  DOutMax=[]  NOutMin=[]  NOutMax=[]  SumOutMin=[]  SumOutMax=[]  SaturationOutMin=[]  SaturationOutMax=[]  PParamMin=[]  PParamMax=[]  IParamMin=[]  IParamMax=[]  DParamMin=[]  DParamMax=[]  NParamMin=[]  NParamMax=[]  KbParamMin=[]  KbParamMax=[]  KtParamMin=[]  KtParamMax=[]  KbOutMin=[]  KbOutMax=[]  KtOutMin=[]  KtOutMax=[]  IntegratorOutMin=[]  IntegratorOutMax=[]  FilterOutMin=[]  FilterOutMax=[]  SumI1OutMin=[]  SumI1OutMax=[]  SumI2OutMin=[]  SumI2OutMax=[]  SumI3OutMin=[]  SumI3OutMax=[]  SumI4OutMin=[]  SumI4OutMax=[]  SumDOutMin=[]  SumDOutMax=[]  DifferentiatorOutMin=[]  DifferentiatorOutMax=[]  FilterDiffOutCoefMin=[]  FilterDiffOutCoefMax=[]  ReciprocalOutMin=[]  ReciprocalOutMax=[]  SumDenOutMin=[]  SumDenOutMax=[]  SumNumOutMin=[]  SumNumOutMax=[]  DivideOutMin=[]  DivideOutMax=[]  UdiffTsProdOutMin=[]  UdiffTsProdOutMax=[]  NTsProdOutMin=[]  NTsProdOutMax=[]  UintegralTsProdOutMin=[]  UintegralTsProdOutMax=[]  UngainTsProdOutMin=[]  UngainTsProdOutMax=[]  ClampingZeroOutDataTypeStr=Inherit: Inherit via back propagation  ClampingZeroOutMin=[]  ClampingZeroOutMax=[]  FilterDenConstantOutDataTypeStr=Inherit: Inherit via back propagation  FilterDenConstantOutMin=[]  FilterDenConstantOutMax=[]  PCopyOutDataTypeStr=Inherit: Inherit via back propagation  PCopyOutMin=[]  PCopyOutMax=[]  NCopyOutDataTypeStr=Inherit: Inherit via back propagation  NCopyOutMin=[]  NCopyOutMax=[]  IntegratorContinuousStateAttributes=''  IntegratorStateMustResolveToSignalObject=off  IntegratorRTWStateStorageClass=Auto  FilterContinuousStateAttributes=''  FilterStateMustResolveToSignalObject=off  FilterRTWStateStorageClass=Auto  ParallelPVariant=InternalParameters  IdealPVariant=Disabled  IVariant=InternalParameters  DVariant=Disabled  IntegratorVariant=Discrete  SatVariant=Enabled  AWVariant=Passthrough  PCopyVariant=Disabled  TRVariant=Disabled  FdbkBlocksVariant=Forward  IdealPFdbkVariant=Disabled  SatFdbkVariant=Disabled  DerivativeFilterVariant=Disabled  NVariant=Disabled  NCopyVariant=Disabled_SignalSpec  FilterICVariant=Disabled  IntegratorICVariant=InternalICs  ExternalResetVariant=Disabled  TRSumVariant=Passthrough  SumFdbkVariant=Disabled  SumVariant=Sum_PI  TsampFilterVariant=InternalTs  TsampNgainVariant=Passthrough  TsampIntegralVariant=Disabled_SignalSpec  ExternalSaturationOutDataTypeStr=Inherit: Same as second input  DerivativeSourceVariant=Disabled  PreIntVariant=InternalPreInt
  Simulink-PS Converter : nesl_utility/Simulink-PS Converter  PhysicalDomain=network_engine_domain  SubClassName=ps_input  LeftPortType=input  RightPortType=output  PseudoPeriodic=off  Frequencies=[]  NoiseDistribution=none  NoiseParameters=[]  Unit=1  AffineConversion=off  FilteringAndDerivatives=provide  SimscapeFilterOrder=1  InputFilterTimeConstant=0.001  UdotUserProvided=0
  Simulink-PS Converter1 : nesl_utility/Simulink-PS Converter  PhysicalDomain=network_engine_domain  SubClassName=ps_input  LeftPortType=input  RightPortType=output  PseudoPeriodic=off  Frequencies=[]  NoiseDistribution=none  NoiseParameters=[]  Unit=1  AffineConversion=off  FilteringAndDerivatives=provide  SimscapeFilterOrder=1  InputFilterTimeConstant=0.001  UdotUserProvided=0
  Subtract : Sum  Inputs=+-
  Subtract1 : Sum  Inputs=+-
  Two-Pulse Gate Multiplexer : ee_lib/Semiconductors & Converters/Converters/Two-Pulse Gate Multiplexer  port_option=ee.enum.controlport.ps
  BATTERY+ : PMIOPort  Side=Left
  BATTERY- : PMIOPort  Port=2  Side=Left
  DC+ : PMIOPort  Port=3  Side=Left
  GROUND : PMIOPort  Port=4  Side=Left
  wires:
  Subtract/1 -> PID Controller/1
  Constant/1 -> Subtract/1
  DC48V/1 -> Subtract/2
  Multiport Switch/1 -> Simulink-PS Converter/1
  Constant2/1 -> Multiport Switch1/4, Multiport Switch1/3
  Constant1/1 -> Multiport Switch/2, Multiport Switch/3
  PID Controller/1 -> Multiport Switch/4
  Subtract1/1 -> PID Controller1/1
  PID Controller1/1 -> Multiport Switch1/2
  I_REFERENCE/1 -> Subtract1/1
  I_BATTERY/1 -> Subtract1/2
  Multiport Switch1/1 -> Simulink-PS Converter1/1
  BATTERY_CMD/1 -> Add/2
  Constant3/1 -> Add/1
  Add/1 -> Multiport Switch1/1, Multiport Switch/1
  connections:
  Bidirectional DC-DC Converter/RConn1 -- BATTERY+/RConn1
  Bidirectional DC-DC Converter/RConn2 -- BATTERY-/RConn1
  DC+/RConn1 -- Bidirectional DC-DC Converter/LConn2
  GROUND/RConn1 -- Bidirectional DC-DC Converter/LConn3
  Two-Pulse Gate Multiplexer/RConn1 -- Bidirectional DC-DC Converter/LConn1
  Simulink-PS Converter/RConn1 -- Two-Pulse Gate Multiplexer/LConn2
  Simulink-PS Converter1/RConn1 -- Two-Pulse Gate Multiplexer/LConn1

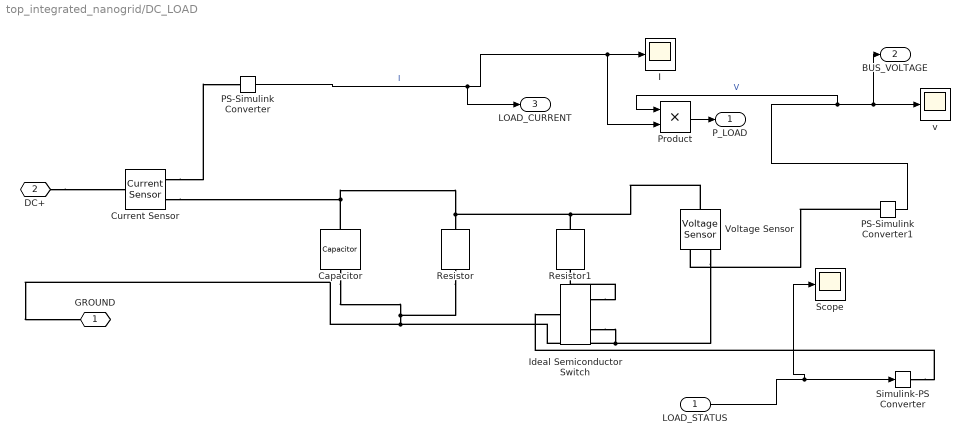
== system top_integrated_nanogrid/DC_LOAD ==
  LOAD_STATUS : Inport
  Capacitor : fl_lib/Electrical/Electrical Elements/Capacitor  c=1000 uF  r=1e-6 Ohm  g=0 1/Ohm  i_specify=on  i_priority=None  i=0 A  i_nominal_specify=off  i_nominal_value=1  i_nominal_unit=A  v_specify=on  v_priority=High  v=48 V  v_nominal_specify=off  v_nominal_value=1  v_nominal_unit=V  vc_specify=on  vc_priority=None  vc=0 V  vc_nominal_specify=off  vc_nominal_value=1  vc_nominal_unit=V
  Current Sensor : fl_lib/Electrical/Electrical Sensors/Current Sensor
  I : Scope
      settings: ActiveDisplayYMinimum=-167.50013113509181  ActiveDisplayYMaximum=39.804090720717255  DataLoggingVariableName=ScopeData21
  Ideal Semiconductor Switch : ee_lib/Semiconductors & Converters/Ideal Semiconductor Switch  port_option=ee.enum.controlport.ps  Ron=0.001 Ohm  Goff=1e-6 1/Ohm  Vth=0.5 V  diode_param=ee.enum.semiconductors.protectionDiode.external  diode_Vf=0.8 V  diode_Ron=0.001 Ohm  diode_Goff=1e-5 1/Ohm  diode_C=50e-9 F  diode_iRM=-235 A  diode_iF=300 A  diode_idot=-50 A/us  diode_trr_param=ee.enum.converters.diodetrr.trr_factor  diode_trr_factor=3  diode_trr=15 us  diode_Qrr=1500 s*uA
  PS-Simulink Converter : nesl_utility/PS-Simulink Converter  PhysicalDomain=network_engine_domain  SubClassName=ps_output  LeftPortType=input  RightPortType=output  PseudoPeriodic=off  Frequencies=[]  VectorFormat=inherit  Unit=inherit  AffineConversion=off
  PS-Simulink Converter1 : nesl_utility/PS-Simulink Converter  PhysicalDomain=network_engine_domain  SubClassName=ps_output  LeftPortType=input  RightPortType=output  PseudoPeriodic=off  Frequencies=[]  VectorFormat=inherit  Unit=inherit  AffineConversion=off
  Product : Product
  Resistor : fl_lib/Electrical/Electrical Elements/Resistor  R=46.08 Ohm  i_specify=off  i_priority=None  i=0 A  i_nominal_specify=off  i_nominal_value=1  i_nominal_unit=A  v_specify=off  v_priority=None  v=0 V  v_nominal_specify=off  v_nominal_value=1  v_nominal_unit=V
  Resistor1 : fl_lib/Electrical/Electrical Elements/Resistor  R=46.08 Ohm  i_specify=off  i_priority=None  i=0 A  i_nominal_specify=off  i_nominal_value=1  i_nominal_unit=A  v_specify=off  v_priority=None  v=0 V  v_nominal_specify=off  v_nominal_value=1  v_nominal_unit=V
  Scope : Scope
      settings: DataLoggingVariableName=ScopeData22
  Simulink-PS Converter : nesl_utility/Simulink-PS Converter  PhysicalDomain=network_engine_domain  SubClassName=ps_input  LeftPortType=input  RightPortType=output  PseudoPeriodic=off  Frequencies=[]  NoiseDistribution=none  NoiseParameters=[]  Unit=1  AffineConversion=off  FilteringAndDerivatives=provide  SimscapeFilterOrder=1  InputFilterTimeConstant=0.001  UdotUserProvided=0
  Voltage Sensor : fl_lib/Electrical/Electrical Sensors/Voltage Sensor
  v : Scope
      settings: ActiveDisplayYMinimum=14.753584599444343  ActiveDisplayYMaximum=59.304634607665662  DataLoggingVariableName=ScopeData23
  GROUND : PMIOPort  Side=Left
  DC+ : PMIOPort  Port=2  Side=Left
  P_LOAD : Outport
  BUS_VOLTAGE : Outport  Port=2
  LOAD_CURRENT : Outport  Port=3
  wires:
  PS-Simulink Converter/1 -> LOAD_CURRENT/1, Product/2, I/1  "I"
  LOAD_STATUS/1 -> Scope/1, Simulink-PS Converter/1
  PS-Simulink Converter1/1 -> Product/1, BUS_VOLTAGE/1, v/1  "V"
  Product/1 -> P_LOAD/1
  connections:
  Resistor1/LConn1 -- Capacitor/LConn1 -- Current Sensor/RConn2 -- Resistor/LConn1 -- Voltage Sensor/LConn1
  Ideal Semiconductor Switch/RConn1 -- Resistor1/RConn1
  Simulink-PS Converter/RConn1 -- Ideal Semiconductor Switch/LConn1
  PS-Simulink Converter1/LConn1 -- Voltage Sensor/RConn1
  Current Sensor/RConn1 -- PS-Simulink Converter/LConn1
  Voltage Sensor/RConn2 -- Ideal Semiconductor Switch/RConn2 -- Resistor/RConn1 -- Capacitor/RConn1 -- GROUND/RConn1
  DC+/RConn1 -- Current Sensor/LConn1

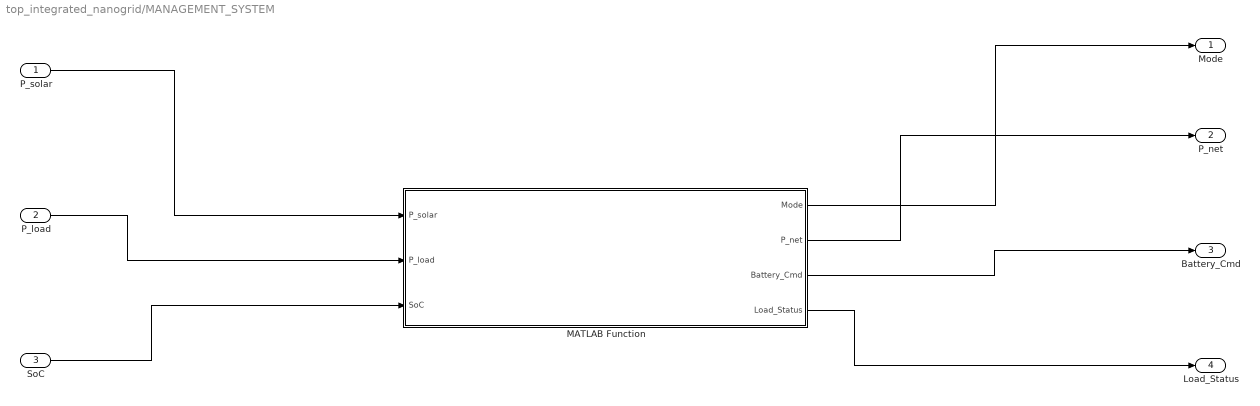
== system top_integrated_nanogrid/MANAGEMENT_SYSTEM ==
  P_solar : Inport
  P_load : Inport  Port=2
  SoC : Inport  Port=3
  MATLAB Function : MATLAB Function  TreatAsAtomicUnit=on
  Mode : Outport
  P_net : Outport  Port=2
  Battery_Cmd : Outport  Port=3
  Load_Status : Outport  Port=4
  wires:
  P_solar/1 -> MATLAB Function/1(P_solar)
  P_load/1 -> MATLAB Function/2(P_load)
  SoC/1 -> MATLAB Function/3(SoC)
  MATLAB Function/1(Mode) -> Mode/1
  MATLAB Function/2(P_net) -> P_net/1
  MATLAB Function/3(Battery_Cmd) -> Battery_Cmd/1
  MATLAB Function/4(Load_Status) -> Load_Status/1

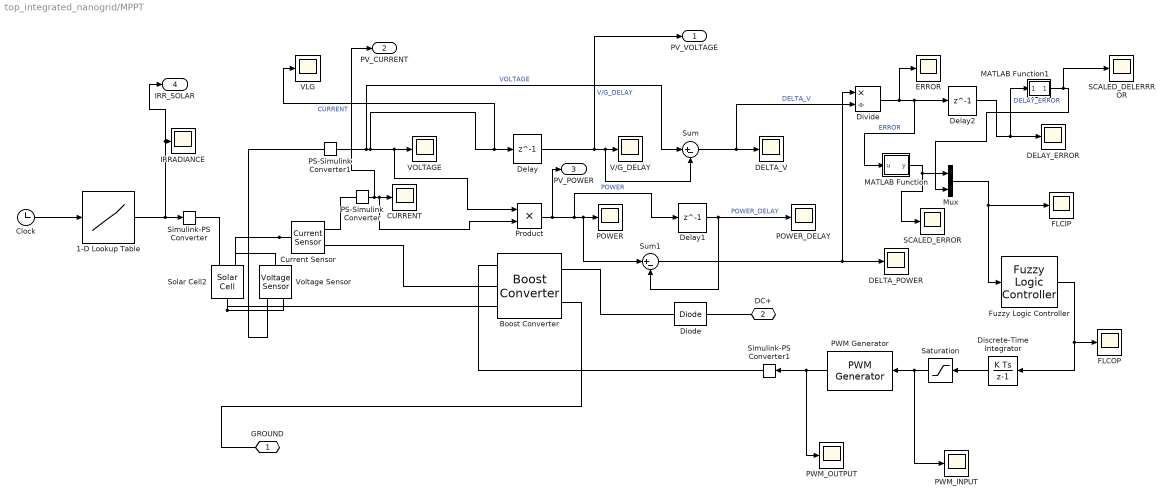
== system top_integrated_nanogrid/MPPT ==
  1-D Lookup Table : Lookup_n-D  NumberOfTableDimensions=1  BreakpointsForDimension1=t_sim  Table=irradiance_day  ExtrapMethod=Clip  InternalRulePriority=Speed  RndMeth=Simplest
  Boost Converter : ee_lib/Semiconductors & Converters/Converters/Boost Converter  port_option=ee.enum.controlport.ps  device_type=ee.enum.converters.switchingdevice.ideal  Vf=0.8 V  Ron=0.001 Ohm  Rds=0.001 Ohm  Goff=1e-5 1/Ohm  Vgt=1 V  Vgt_off=-1 V  Ih=1 A  Vth=6 V  K=0  diode_param=ee.enum.converters.protectiondiode.nodynamics  diode_Vf=0.8 V  diode_Ron=0.001 Ohm  diode_Goff=1e-5 1/Ohm  diode_C=50 nF  diode_iRM=-235 A  diode_iF=300 A  diode_idot=-50 A/us  diode_trr_param=ee.enum.converters.diodetrr.trr_factor  diode_trr_factor=3  diode_trr=15 us  diode_Qrr=1500 s*uA  Lf=1e-6 H  Rl=0 Ohm  Cf=1e-7 F  Rf=1e-6 Ohm  snubber_type=ee.enum.converters.snubber.exclude  Cs=1e-7 F  Rs=0.1 Ohm  iL_specify=off  iL_priority=High  iL=0 A  iL_nominal_specify=off  iL_nominal_value=1  iL_nominal_unit=A  vc_specify=off  vc_priority=High  vc=0 V  vc_nominal_specify=off  vc_nominal_value=1  vc_nominal_unit=V
  CURRENT : Scope
      settings: ActiveDisplayYMinimum=-0.41356913543245555  ActiveDisplayYMaximum=3.72159786600263
  Clock : Clock
  Current Sensor : fl_lib/Electrical/Electrical Sensors/Current Sensor
  DELAY_ERROR : Scope
      settings: ActiveDisplayYMinimum=-1  ActiveDisplayYMaximum=1  DataLoggingVariableName=ScopeData8
  DELTA_POWER : Scope
      settings: DataLoggingVariableName=ScopeData6
  DELTA_V : Scope
      settings: DataLoggingVariableName=ScopeData3
  Delay : Delay  DelayLength=1  InputProcessing=Columns as channels (frame based)
  Delay1 : Delay  DelayLength=1  InputProcessing=Columns as channels (frame based)
  Delay2 : Delay  DelayLength=1  InputProcessing=Columns as channels (frame based)
  Diode : ee_lib/Semiconductors & Converters/Diode  ModelType=ee.enum.diode.modelType.pwl  TableType=ee.enum.diode.tableType.IfMat  IfMat=[.07, .12, .19, 1.75, 4.24, 7.32, 11.2; .16, .3, .72, 2.14, 5.02, 8.35, 13.12] A  VfMat=[.9, 1.15, 1.25, 1.5, 1.75, 2.17, 2.6, 2.85; .58, .68, .75, 1.1, 1.38, 1.77, 2.27, 2.7] V  TjVec=[25, 125] degC  VfVec=[.5, .7, .9, 1.3, 1.7, 2.1, 2.5] V  IfVec=[.1, .2, .5, 1, 2, 4, 7, 10] A  IrMat=[1e-06, 2e-06, 5e-06, 1e-05, 2.5e-05, 5e-05, .0001; 2e-06, 5e-06, 1e-05, 4e-05, 8e-05, .0002, .0005] A  VrMat=[10, 100, 200, 250, 300, 325, 350; 10, 70, 160, 220, 270, 300, 320] V  VrVec=[10, 20, 40, 50, 70, 80, 100] V  IrVec=[1e-06, 2e-06, 5e-06, 1e-05, 2e-05, 5e-05, .0001] A  Vf=0.6 V  Ron=0.3 Ohm  Goff=1e-8 S  prmExp=ee.enum.diode.expParam.useTwo  I12=[.0137, .545] A  V12=[.6, .7] V  RS=0 Ohm  Tmeas=298.15 K  IS=1e-12 A  ec=1  I1=0.0137 A  V1=0.6 V  N_series=1  N_parallel=1  ZenerEnable=false  Rz=0.3 Ohm  BV=30 V  C_param=ee.enum.diode.capParam.fixed  CJ=0 pF  CJ0=5 pF  Vvec=[.1, 10, 100] V  Cvec=[3.5, 1, .4] pF  VJ=1 V  Mgrad=0.5  FC=0.5  Q_param=ee.enum.diode.recoveryParam.off  iRM=-7.15 A  iF=4 A  didt=-750 A/us  trr_factor=3  trr=115 ns  Qrr=150 nA*s  Vr=-600 V  Ls=150 nH  Erec=0.03 J  TT=50 ns  tau=100 ns  T_param=ee.enum.diode.temperatureParam.off  Tdevice=298.15 K  I1_T2=0.245 A  V1_T2=0.5 V  IS_T2=1.25e-7 A  Tmeas2=125 degC  XTI_param=ee.enum.diode.xtiParam.pn  XTI=3  EG_param=ee.enum.diode.egapParam.material_si  EG=1.11 eV  dBVdT=0 V/K  enable_fault_input=simscape.enum.onoff.off  i_specify=off  i_priority=None  i=0 A  i_nominal_specify=off  i_nominal_value=1  i_nominal_unit=A  v_specify=off  v_priority=None  v=0 V  v_nominal_specify=off  v_nominal_value=1  v_nominal_unit=V  v_capacitor_specify=off  v_capacitor_priority=None  v_capacitor=0 V  v_capacitor_nominal_specify=off  v_capacitor_nominal_value=1  v_capacitor_nominal_unit=V  Qj_specify=off  Qj_priority=High  Qj=0 C  Qj_nominal_specify=off  Qj_nominal_value=1  Qj_nominal_unit=C  i_diode_specify=off  i_diode_priority=None  i_diode=0 A  i_diode_nominal_specify=off  i_diode_nominal_value=1  i_diode_nominal_unit=A  v_diode_specify=off  v_diode_priority=None  v_diode=0 V  v_diode_nominal_specify=off  v_diode_nominal_value=1  v_diode_nominal_unit=V  i_capacitor_specify=off  i_capacitor_priority=None  i_capacitor=0 A  i_capacitor_nominal_specify=off  i_capacitor_nominal_value=1  i_capacitor_nominal_unit=A  fidelity_level=ee.enum.diode.fidelity.includeChargeDyn  rec_loss_model=ee.enum.diode.reverseRecoveryModelTabulateUpTo3D.fixed  ErecVal=0 J  scaleWithIandV=true  ErecMat=zeros(2, 3) J  ErecMat3D=zeros(2, 3, 2) J  TjrecVec=[298.15, 398.15] K  IfrecVec=[.1, 1, 10] A  IrecVal=10 A  VrecVal=10 V  VrecVec=[0, 100] V  tFilter=1 / 1000 / 100 s  thermal_network_parameterization=ee.enum.thermalNetworkTopology.junctionCase  Rth=[0, 10] K/W  Rth_Cauer=[1, 3, 10] K/W  Rth_Foster=[.08, .14, .22, .16] K/W  thermal_mass_parameterization=ee.enum.thermalNetwork.timeconstant  thermal_mass=[0, 1] J/K  thermal_mass_Cauer=[.1, .3, 1] J/K  thermal_mass_Foster=[.001, .005, .05, .5] J/K  thermal_time_constant=[0, 10] s  thermal_time_constant_Cauer=[1, 3, 10] s  thermal_time_constant_Foster=[7e-05, .0007, .01, .08] s  thermal_mass_initial_temperatures=[25, 25] degC  thermal_mass_initial_temperatures_Cauer=[25, 25, 25] degC  junction_thermal_mass=0.01 J/K  Tvec_initial_Foster=[25, 25, 25, 25] degC  no_thermal_network=0  junction_temperature_specify=off  junction_temperature_priority=None  junction_temperature=25 degC  junction_temperature_nominal_specify=off  junction_temperature_nominal_value=1  junction_temperature_nominal_unit=degC
  Discrete-Time Integrator : DiscreteIntegrator  InitialCondition=0.4  SampleTime=-1  ICPrevOutput=DiscIntNeverNeededParam  ICPrevScaledInput=DiscIntNeverNeededParam
  Divide : Product  Inputs=*/
  ERROR : Scope
      settings: ActiveDisplayYMinimum=-1  ActiveDisplayYMaximum=1  DataLoggingVariableName=ScopeData7
  FLCIP : Scope
      settings: ActiveDisplayYMinimum=-1  ActiveDisplayYMaximum=1  DataLoggingVariableName=ScopeData10
  FLCOP : Scope
      settings: ActiveDisplayYMinimum=-1  ActiveDisplayYMaximum=1  DataLoggingVariableName=ScopeData9
  Fuzzy Logic Controller : fuzblock/Fuzzy Logic  Controller  FIS=mppt_fuzzy  OutputSampleNumber=101  DataType=double  UseLookupTable=off  NumBreakpoints=10  FuzzifiedInputs=off  RuleFiringStrengths=off  RuleOutputs=off  AggregatedOutputs=off  SimulateUsing=Interpreted execution  OutOfRangeInputValueMessage=warning  NoRuleFiredMessage=warning  EmptyOutputFuzzySetMessage=warning
  IRRADIANCE : Scope
      settings: ActiveDisplayYMinimum=-1  ActiveDisplayYMaximum=1  DataLoggingVariableName=ScopeData16
  MATLAB Function : MATLAB Function  TreatAsAtomicUnit=on
  MATLAB Function1 : MATLAB Function  TreatAsAtomicUnit=on
  Mux : Mux  Inputs=2
  POWER : Scope
      settings: ActiveDisplayYMinimum=-8.159722551352943E-14  ActiveDisplayYMaximum=9.0663583903921573E-15  DataLoggingVariableName=ScopeData4
  POWER_DELAY : Scope
      settings: ActiveDisplayYMinimum=-14.00862484680504  ActiveDisplayYMaximum=126.07762362109794  DataLoggingVariableName=ScopeData5
  PS-Simulink Converter : nesl_utility/PS-Simulink Converter  PhysicalDomain=network_engine_domain  SubClassName=ps_output  LeftPortType=input  RightPortType=output  PseudoPeriodic=off  Frequencies=[]  VectorFormat=inherit  Unit=inherit  AffineConversion=off
  PS-Simulink Converter1 : nesl_utility/PS-Simulink Converter  PhysicalDomain=network_engine_domain  SubClassName=ps_output  LeftPortType=input  RightPortType=output  PseudoPeriodic=off  Frequencies=[]  VectorFormat=inherit  Unit=inherit  AffineConversion=off
  PWM Generator : eePwmGenerator/PWM Generator  CarrCount=Up  Tper=0.001  Tdelay=0  Ts=5e-5
  PWM_INPUT : Scope
      settings: ActiveDisplayYMinimum=-1  ActiveDisplayYMaximum=1  DataLoggingVariableName=ScopeData12
  PWM_OUTPUT : Scope
      settings: ActiveDisplayYMinimum=-1  ActiveDisplayYMaximum=1  DataLoggingVariableName=ScopeData11
  Product : Product
  SCALED_DELERRROR : Scope
      settings: ActiveDisplayYMinimum=-1  ActiveDisplayYMaximum=1  DataLoggingVariableName=ScopeData14
  SCALED_ERROR : Scope
      settings: ActiveDisplayYMinimum=-1  ActiveDisplayYMaximum=1  DataLoggingVariableName=ScopeData13
  Saturation : Saturate  UpperLimit=0.9  LowerLimit=0.05
  Simulink-PS Converter : nesl_utility/Simulink-PS Converter  PhysicalDomain=network_engine_domain  SubClassName=ps_input  LeftPortType=input  RightPortType=output  PseudoPeriodic=off  Frequencies=[]  NoiseDistribution=none  NoiseParameters=[]  Unit=1  AffineConversion=off  FilteringAndDerivatives=provide  SimscapeFilterOrder=1  InputFilterTimeConstant=0.001  UdotUserProvided=0
  Simulink-PS Converter1 : nesl_utility/Simulink-PS Converter  PhysicalDomain=network_engine_domain  SubClassName=ps_input  LeftPortType=input  RightPortType=output  PseudoPeriodic=off  Frequencies=[]  NoiseDistribution=none  NoiseParameters=[]  Unit=1  AffineConversion=off  FilteringAndDerivatives=provide  SimscapeFilterOrder=1  InputFilterTimeConstant=0.001  UdotUserProvided=0
  Solar Cell2 : ee_lib/Sources/Solar Cell  prm=ee.enum.sources.solar_cell_prm.eightParameter  Isc=7.34 A  Voc=21.5 V  Is=1e-10 A  Is2=1e-10 A  Iph=7.34 A  Ir0=1000 W/m^2  ec=1.5  N2=2  Rs=0 Ohm  Rp=inf Ohm  N_series=36  N_parallel=1  TIPH1=0 1/K  EG=1.11 eV  TXIS1=3  TXIS2=3  TRS1=0  TRP1=0  Tmeas=25 degC  TFIXED=25 degC  thermal_mass=100 J/K  initial_temperature=25 degC
  Sum : Sum  Inputs=|+-
  Sum1 : Sum  Inputs=|+-
  V/G_DELAY : Scope
      settings: ActiveDisplayYMinimum=0.013867681033747642  ActiveDisplayYMaximum=0.03386768103374764  DataLoggingVariableName=ScopeData2
  VLG : Scope
      settings: ActiveDisplayYMinimum=-130444.09260685327  ActiveDisplayYMaximum=14531.429559128628  DataLoggingVariableName=ScopeData15
  VOLTAGE : Scope
      settings: ActiveDisplayYMinimum=-1  ActiveDisplayYMaximum=1
  Voltage Sensor : fl_lib/Electrical/Electrical Sensors/Voltage Sensor
  GROUND : PMIOPort  Side=Left
  DC+ : PMIOPort  Port=2  Side=Right
  PV_VOLTAGE : Outport
  PV_CURRENT : Outport  Port=2
  PV_POWER : Outport  Port=3
  IRR_SOLAR : Outport  Port=4
  wires:
  Saturation/1 -> PWM_INPUT/1, PWM Generator/1
  Fuzzy Logic Controller/1 -> FLCOP/1, Discrete-Time Integrator/1
  Sum1/1 -> Divide/1, DELTA_POWER/1
  Mux/1 -> FLCIP/1, Fuzzy Logic Controller/1
  Sum/1 -> Divide/2, DELTA_V/1  "DELTA_V"
  MATLAB Function/1(y) -> SCALED_ERROR/1, Mux/1
  PWM Generator/1 -> PWM_OUTPUT/1, Simulink-PS Converter1/1
  Discrete-Time Integrator/1 -> Saturation/1
  PS-Simulink Converter/1 -> PV_CURRENT/1, Product/2, CURRENT/1  "CURRENT"
  MATLAB Function1/1(y) -> SCALED_DELERRROR/1, Mux/2
  Delay/1 -> PV_VOLTAGE/1, Sum/2, V/G_DELAY/1  "V/G_DELAY"
  Divide/1 -> ERROR/1, MATLAB Function/1(u), Delay2/1  "ERROR"
  Delay2/1 -> MATLAB Function1/1(u), DELAY_ERROR/1  "DELAY_ERROR"
  Clock/1 -> 1-D Lookup Table/1
  PS-Simulink Converter1/1 -> Sum/1, VLG/1, Delay/1, Product/1, VOLTAGE/1  "VOLTAGE"
  Delay1/1 -> Sum1/2, POWER_DELAY/1  "POWER_DELAY"
  1-D Lookup Table/1 -> IRR_SOLAR/1, IRRADIANCE/1, Simulink-PS Converter/1
  Product/1 -> PV_POWER/1, Delay1/1, Sum1/1, POWER/1  "POWER"
  connections:
  GROUND/RConn1 -- Boost Converter/RConn2
  Current Sensor/LConn1 -- Solar Cell2/LConn2 -- Voltage Sensor/LConn1
  Voltage Sensor/RConn2 -- Solar Cell2/RConn1 -- Boost Converter/LConn3
  Current Sensor/RConn1 -- PS-Simulink Converter/LConn1
  Simulink-PS Converter1/RConn1 -- Boost Converter/LConn1
  Voltage Sensor/RConn1 -- PS-Simulink Converter1/LConn1
  Current Sensor/RConn2 -- Boost Converter/LConn2
  Diode/LConn1 -- Boost Converter/RConn1
  Simulink-PS Converter/RConn1 -- Solar Cell2/LConn1
  DC+/RConn1 -- Diode/RConn1

== matlab function top_integrated_nanogrid/MPPT/MATLAB Function1 ==
  data: u input; y output
function y = scale_angle(u)
    y = u / 180;
end
